simulink model "gm_HFMA_4B_1_5_9_13"  (R2026b)
settings: Solver=FixedStepDiscrete  StopTime=stopTime  FixedStep=1.953125e-06
PreLoadFcn:
  | load('a_luts.mat')
undefined symbols (not defined in the file or in its folder): Ts
libraries: simulink x202, simulink_need_slupdate x99, hdlsllib x91
(part 1 of 20)
settings Model: FPTRunName=BaselineRun  Creator=Kayla  LastModifiedBy=Kayla
settings OptimizationCC: BlockReduction=off  ConditionallyExecuteInputs=off  DefaultParameterBehavior=Inlined  InheritOutputTypeSmallerThanSingle=on
settings DebuggingCC: ArtificialAlgebraicLoopMsg=error  InheritedTsInSrcMsg=none  IntegerOverflowMsg=none  IntegerSaturationMsg=none  ParameterPrecisionLossMsg=none  SignalRangeChecking=warning  SingleTaskRateTransMsg=error
settings HardwareCC: ProdEndianess=Unspecified  ProdEqTarget=off  ProdHWDeviceType=ASIC/FPGA->ASIC/FPGA  ProdIntDivRoundTo=Undefined  ProdLargestAtomicFloat=None  TargetEndianess=LittleEndian  TargetHWDeviceType=Custom Processor->MATLAB Host Computer  TargetIntDivRoundTo=Zero  TargetLongLongMode=on

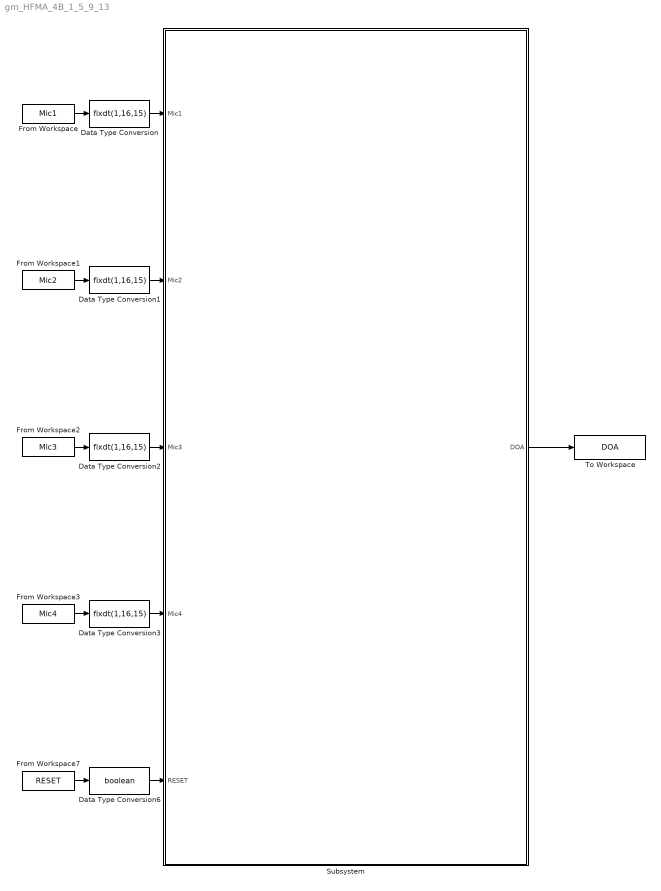
== system gm_HFMA_4B_1_5_9_13 ==
  Data Type Conversion{,1..3} (4 alike) : DataTypeConversion  OutDataTypeStr=fixdt(1,16,15)  RndMeth=Nearest
  Data Type Conversion6 : DataTypeConversion  OutDataTypeStr=boolean  RndMeth=Nearest
  From Workspace : FromWorkspace  VariableName=Mic1  SampleTime=Ts  Interpolate=off  OutputAfterFinalValue=Holding final value
  From Workspace1 : FromWorkspace  VariableName=Mic2  SampleTime=Ts  Interpolate=off  OutputAfterFinalValue=Holding final value
  From Workspace2 : FromWorkspace  VariableName=Mic3  SampleTime=Ts  Interpolate=off  OutputAfterFinalValue=Holding final value
  From Workspace3 : FromWorkspace  VariableName=Mic4  SampleTime=Ts  Interpolate=off  OutputAfterFinalValue=Holding final value
  From Workspace7 : FromWorkspace  VariableName=RESET  SampleTime=Ts
  Subsystem : Subsystem
  To Workspace : ToWorkspace  VariableName=DOA  SaveFormat=Timeseries  SampleTime=-1
  wires:
  Data Type Conversion6/1 -> Subsystem/5(RESET)
  Data Type Conversion3/1 -> Subsystem/4(Mic4)
  Data Type Conversion2/1 -> Subsystem/3(Mic3)
  Data Type Conversion1/1 -> Subsystem/2(Mic2)
  Data Type Conversion/1 -> Subsystem/1(Mic1)
  From Workspace3/1 -> Data Type Conversion3/1
  From Workspace2/1 -> Data Type Conversion2/1
  From Workspace1/1 -> Data Type Conversion1/1
  From Workspace/1 -> Data Type Conversion/1
  Subsystem/1(DOA) -> To Workspace/1
  From Workspace7/1 -> Data Type Conversion6/1
